simulink library "Driver_Glider_Library"  (R2017b)
settings: Solver=VariableStepAuto  StartTime=0.0  StopTime=10.0  RelTol=1e-3
undefined symbols (not defined in the file or in its folder): aeroDragCoeff, airDensity, frontArea, gravity, inclinationAngle, inertialMassVeh, magnitude, massVeh, rollingResistCoeff
libraries: simulink x1
settings Model: Creator=emarquez  LastModifiedBy=emarquez
settings CodeAppCC: StateflowObjectComments=on

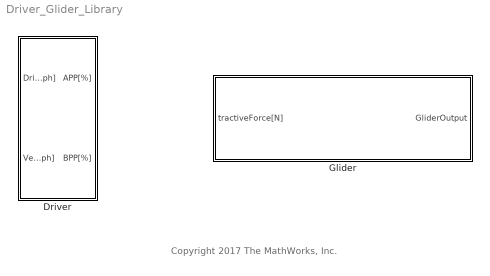
== system Driver_Glider_Library ==
  note: Copyright 2017 The MathWorks, Inc.
  Driver : Subsystem
      mask Display: image('DriverPic.jpg');
  Glider : Subsystem
      mask Display: image('VehiclePic.jpg');

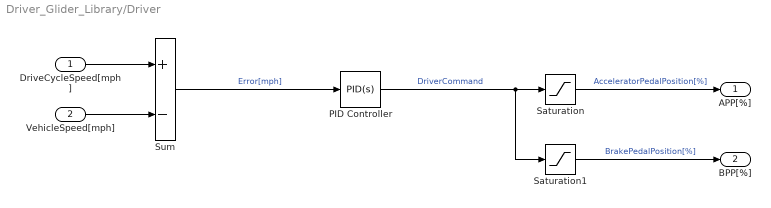
== system Driver_Glider_Library/Driver ==
  DriveCycleSpeed[mph] : Inport
  VehicleSpeed[mph] : Inport  Port=2
  PID Controller : simulink/Continuous/PID Controller  Controller=PID  TimeDomain=Continuous-time  SampleTime=-1  IntegratorMethod=Forward Euler  FilterMethod=Forward Euler  Form=Parallel  UseFilter=on  ControllerParametersSource=internal  P=250  I=1  D=0  N=100  InitialConditionSource=internal  InitialConditionForIntegrator=0  InitialConditionForFilter=0  ExternalReset=none  LimitOutput=off  UpperSaturationLimit=inf  LowerSaturationLimit=-inf  LinearizeAsGain=on  AntiWindupMode=none  Kb=1  TrackingMode=off  Kt=1  PParamMin=[]  PParamMax=[]  IParamMin=[]  IParamMax=[]  DParamMin=[]  DParamMax=[]  NParamMin=[]  NParamMax=[]  KbParamMin=[]  KbParamMax=[]  KtParamMin=[]  KtParamMax=[]  POutMin=[]  POutMax=[]  IOutMin=[]  IOutMax=[]  DOutMin=[]  DOutMax=[]  NOutMin=[]  NOutMax=[]  KbOutMin=[]  KbOutMax=[]  KtOutMin=[]  KtOutMax=[]  IntegratorOutMin=[]  IntegratorOutMax=[]  FilterOutMin=[]  FilterOutMax=[]  SumOutMin=[]  SumOutMax=[]  SumI1OutMin=[]  SumI1OutMax=[]  SumI2OutMin=[]  SumI2OutMax=[]  SumI3OutMin=[]  SumI3OutMax=[]  SumDOutMin=[]  SumDOutMax=[]  SaturationOutMin=[]  SaturationOutMax=[]  IntegratorContinuousStateAttributes=''  IntegratorStateMustResolveToSignalObject=off  IntegratorRTWStateStorageClass=Auto  FilterContinuousStateAttributes=''  FilterStateMustResolveToSignalObject=off  FilterRTWStateStorageClass=Auto  DifferentiatorICPrevScaledInput=0  DifferentiatorOutMin=[]  DifferentiatorOutMax=[]  InitialConditionSetting=State (most efficient)
  Saturation : Saturate  UpperLimit=100  LowerLimit=0  ZeroCross=off
  Saturation1 : Saturate  UpperLimit=0  LowerLimit=-100  ZeroCross=off
  Sum : Sum  Inputs=+-
  APP[%] : Outport
  BPP[%] : Outport  Port=2
  wires:
  VehicleSpeed[mph]/1 -> Sum/2
  Sum/1 -> PID Controller/1  "Error[mph]"
  Saturation1/1 -> BPP[%]/1  "BrakePedalPosition[%]"
  PID Controller/1 -> Saturation/1, Saturation1/1  "DriverCommand"
  Saturation/1 -> APP[%]/1  "AcceleratorPedalPosition[%]"
  DriveCycleSpeed[mph]/1 -> Sum/1

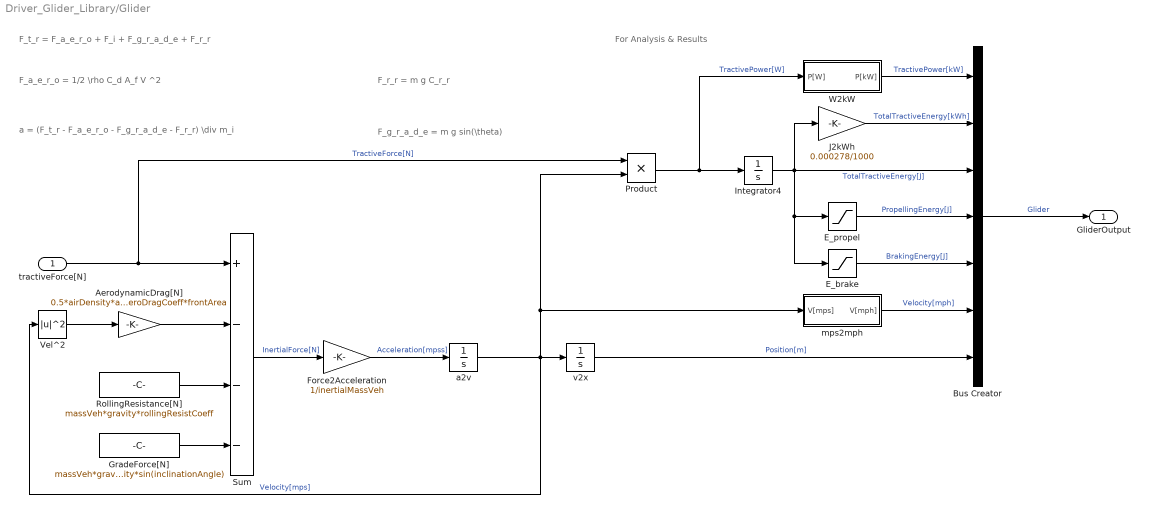
== system Driver_Glider_Library/Glider ==
  note: F_g_r_a_d_e = m g sin(\theta)
  note: F_a_e_r_o = 1/2 \rho C_d A_f V ^2
  note: For Analysis & Results
  note: F_r_r = m g C_r_r
  note: a = (F_t_r - F_a_e_r_o - F_g_r_a_d_e - F_r_r) \div m_i
  note: F_t_r = F_a_e_r_o + F_i + F_g_r_a_d_e + F_r_r
  tractiveForce[N] : Inport
  AerodynamicDrag[N] : Gain  Gain=0.5*airDensity*aeroDragCoeff*frontArea
      settings: AttributesFormatString=%<Gain>
  Bus Creator : BusCreator  Inputs=7
  E_brake : Saturate  UpperLimit=0  LowerLimit=-inf
  E_propel : Saturate  UpperLimit=inf  LowerLimit=0
  Force2Acceleration : Gain  Gain=1/inertialMassVeh
      settings: AttributesFormatString=%<Gain>
  GradeForce[N] : Constant  Value=massVeh*gravity*sin(inclinationAngle)
      settings: AttributesFormatString=%<Value>
  Integrator4 : Integrator
  J2kWh : Gain  Gain=0.000278/1000
  Product : Product
  RollingResistance[N] : Constant  Value=massVeh*gravity*rollingResistCoeff
      settings: AttributesFormatString=%<Value>
  Sum : Sum  Inputs=+---
  Vel^2 : Math  Operator=magnitude^2  SaturateOnIntegerOverflow=on
  W2kW : Subsystem
  a2v : Integrator
  mps2mph : Subsystem
  v2x : Integrator
  GliderOutput : Outport
  wires:
  Bus Creator/1 -> GliderOutput/1  "Glider"
  Product/1 -> Integrator4/1, W2kW/1(P[W])  "TractivePower[W]"
  tractiveForce[N]/1 -> Sum/1, Product/1  "TractiveForce[N]"
  a2v/1 -> Product/2, mps2mph/1(V[mps]), Vel^2/1, v2x/1  "Velocity[mps]"
  v2x/1 -> Bus Creator/7  "Position[m]"
  AerodynamicDrag[N]/1 -> Sum/2
  GradeForce[N]/1 -> Sum/4
  RollingResistance[N]/1 -> Sum/3
  E_brake/1 -> Bus Creator/5  "BrakingEnergy[J]"
  Force2Acceleration/1 -> a2v/1  "Acceleration[mpss]"
  Integrator4/1 -> E_propel/1, E_brake/1, Bus Creator/3, J2kWh/1  "TotalTractiveEnergy[J]"
  Vel^2/1 -> AerodynamicDrag[N]/1
  W2kW/1(P[kW]) -> Bus Creator/1  "TractivePower[kW]"
  E_propel/1 -> Bus Creator/4  "PropellingEnergy[J]"
  mps2mph/1(V[mph]) -> Bus Creator/6  "Velocity[mph]"
  Sum/1 -> Force2Acceleration/1  "InertialForce[N]"
  J2kWh/1 -> Bus Creator/2  "TotalTractiveEnergy[kWh]"

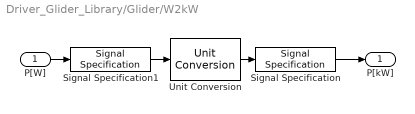
== system Driver_Glider_Library/Glider/W2kW ==
  P[W] : Inport
  Signal Specification : SignalSpecification  Unit=kW
  Signal Specification1 : SignalSpecification  Unit=W
  Unit Conversion : UnitConversion
  P[kW] : Outport
  wires:
  P[W]/1 -> Signal Specification1/1
  Unit Conversion/1 -> Signal Specification/1
  Signal Specification1/1 -> Unit Conversion/1
  Signal Specification/1 -> P[kW]/1

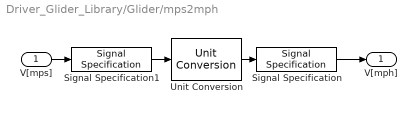
== system Driver_Glider_Library/Glider/mps2mph ==
  V[mps] : Inport
  Signal Specification : SignalSpecification  Unit=mph
  Signal Specification1 : SignalSpecification  Unit=m/s
  Unit Conversion : UnitConversion
  V[mph] : Outport
  wires:
  Signal Specification/1 -> V[mph]/1
  Signal Specification1/1 -> Unit Conversion/1
  Unit Conversion/1 -> Signal Specification/1
  V[mps]/1 -> Signal Specification1/1
